simulink subsystem "dq_Limiter"  (R2022b)
settings: Solver=VariableStepAuto  StartTime=0.0  StopTime=10.0  RelTol=1e-3
model mask{X_dq_max=1, limType=Constant ratio d/q, datatype='double'}
  mask prompts: datatype "Signal data type"
libraries: simulink x5
settings Model: Creator=winkens  LastModifiedBy=winkens
settings SolverCC: AlgebraicLoopSolver=TrustRegion
settings DebuggingCC: UnconnectedInputMsg=warning  UnconnectedOutputMsg=warning  UnconnectedLineMsg=warning  SFMachineParentedDataDiag=warning
settings ModelReferenceCC: EnableRefExpFcnMdlSchedulingChecks=on
settings RTWCC: DLArmComputeVersion=19.05

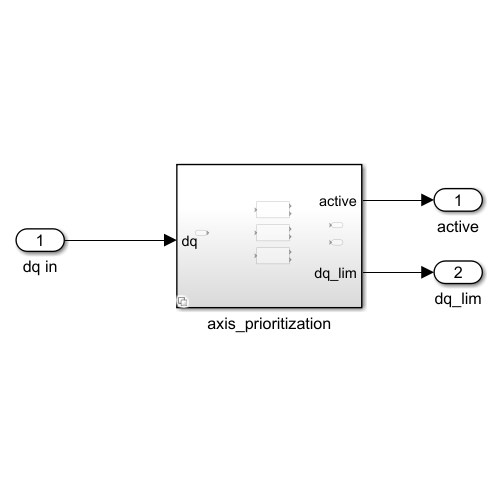
[thumbnail: Simulink's stored preview of the top-level diagram]
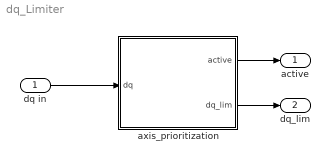
== system dq_Limiter ==
  dq in : Inport
  axis_prioritization : Subsystem  Variant=on
  active : Outport
  dq_lim : Outport  Port=2
  wires:
  dq in/1 -> axis_prioritization/1(dq)
  axis_prioritization/2(dq_lim) -> dq_lim/1
  axis_prioritization/1(active) -> active/1

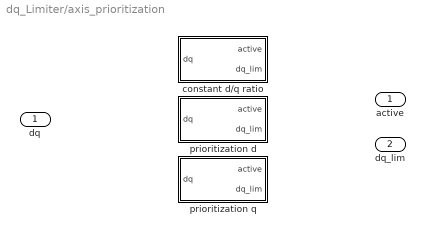
== system dq_Limiter/axis_prioritization ==
  dq : Inport
  constant d/q ratio : Subsystem  VariantControl=(default)
  prioritization d : Subsystem  VariantControl=limType == 2
  prioritization q : Subsystem  VariantControl=limType == 3
  active : Outport  OutDataTypeStr=boolean
  dq_lim : Outport  Port=2

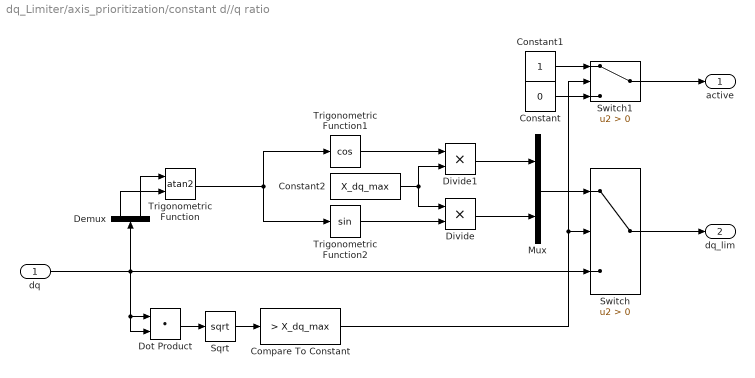
== system dq_Limiter/axis_prioritization/constant d//q ratio ==
  dq : Inport
  Compare To Constant : simulink/Logic and Bit Operations/Compare To Constant  relop=>  const=X_dq_max  OutDataTypeStr=boolean
  Constant : Constant  Value=0  OutDataTypeStr=boolean
  Constant1 : Constant  OutDataTypeStr=boolean
  Constant2 : Constant  Value=X_dq_max  OutDataTypeStr=datatype
  Demux : Demux  Outputs=2
  Divide : Product  Inputs=**
  Divide1 : Product  Inputs=**
  Dot Product : DotProduct  OutDataTypeStr=Inherit: Inherit via internal rule
  Mux : Mux  Inputs=2
  Sqrt : Sqrt
  Switch : Switch  Criteria=u2 > Threshold  SaturateOnIntegerOverflow=off  InputSameDT=off
  Switch1 : Switch  Criteria=u2 > Threshold  SaturateOnIntegerOverflow=off  InputSameDT=off
  Trigonometric Function : Trigonometry  Operator=atan2
  Trigonometric Function1 : Trigonometry  Operator=cos
  Trigonometric Function2 : Trigonometry
  active : Outport  OutDataTypeStr=boolean
  dq_lim : Outport  Port=2
  wires:
  Trigonometric Function/1 -> Trigonometric Function2/1, Trigonometric Function1/1
  Trigonometric Function1/1 -> Divide1/1
  Trigonometric Function2/1 -> Divide/2
  Constant2/1 -> Divide1/2, Divide/1
  Divide/1 -> Mux/2
  Divide1/1 -> Mux/1
  Mux/1 -> Switch/1
  Demux/1 -> Trigonometric Function/2
  Demux/2 -> Trigonometric Function/1
  Compare To Constant/1 -> Switch/2, Switch1/2
  Dot Product/1 -> Sqrt/1
  Switch1/1 -> active/1
  Constant1/1 -> Switch1/1
  Constant/1 -> Switch1/3
  Sqrt/1 -> Compare To Constant/1
  Switch/1 -> dq_lim/1
  dq/1 -> Demux/1, Switch/3, Dot Product/2, Dot Product/1

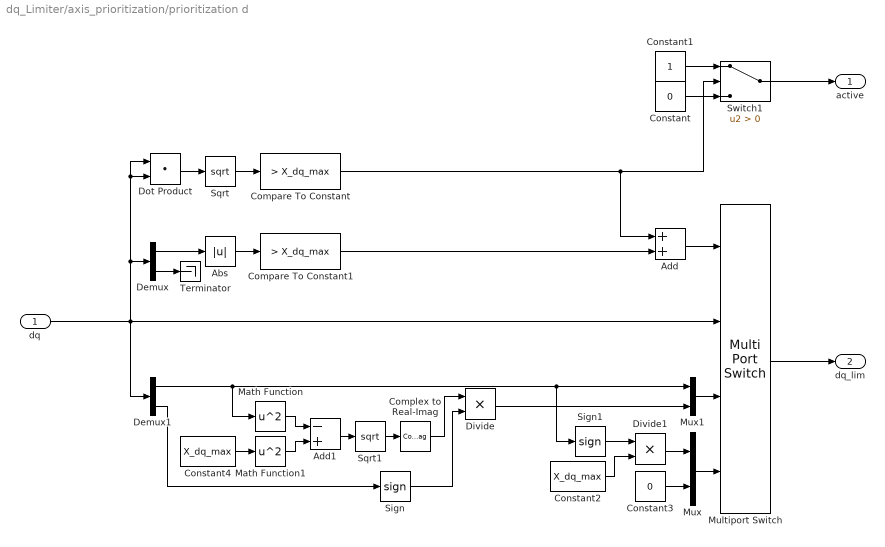
== system dq_Limiter/axis_prioritization/prioritization d ==
  dq : Inport
  Abs : Abs  SaturateOnIntegerOverflow=off
  Add : Sum
  Add1 : Sum  Inputs=-+
  Compare To Constant : simulink/Logic and Bit Operations/Compare To Constant  relop=>  const=X_dq_max  OutDataTypeStr=uint8
  Compare To Constant1 : simulink/Logic and Bit Operations/Compare To Constant  relop=>  const=X_dq_max  OutDataTypeStr=uint8
  Complex to Real-Imag : ComplexToRealImag  Output=Real
  Constant : Constant  Value=0  OutDataTypeStr=boolean
  Constant1 : Constant  OutDataTypeStr=boolean
  Constant2 : Constant  Value=X_dq_max  OutDataTypeStr=datatype
  Constant3 : Constant  Value=0  OutDataTypeStr=datatype
  Constant4 : Constant  Value=X_dq_max  OutDataTypeStr=datatype
  Demux : Demux  Outputs=2
  Demux1 : Demux  Outputs=2
  Divide : Product  Inputs=**
  Divide1 : Product  Inputs=**
  Dot Product : DotProduct  OutDataTypeStr=Inherit: Inherit via internal rule
  Math Function : Math  Operator=square
  Math Function1 : Math  Operator=square
  Multiport Switch : MultiPortSwitch  DataPortOrder=Zero-based contiguous  zeroidx=on  SaturateOnIntegerOverflow=off  InputSameDT=off
  Mux : Mux  Inputs=2
  Mux1 : Mux  Inputs=2
  Sign : Signum
  Sign1 : Signum
  Sqrt : Sqrt
  Sqrt1 : Sqrt  OutputSignalType=complex
  Switch1 : Switch  Criteria=u2 > Threshold  SaturateOnIntegerOverflow=off  InputSameDT=off
  Terminator : Terminator
  active : Outport  OutDataTypeStr=boolean
  dq_lim : Outport  Port=2
  wires:
  Sign1/1 -> Divide1/1
  Constant2/1 -> Divide1/2
  Abs/1 -> Compare To Constant1/1
  Complex to Real-Imag/1 -> Divide/1
  Sqrt1/1 -> Complex to Real-Imag/1
  Sign/1 -> Divide/2
  Divide/1 -> Mux1/2
  Add1/1 -> Sqrt1/1
  Math Function1/1 -> Add1/2
  Math Function/1 -> Add1/1
  Constant4/1 -> Math Function1/1
  Demux1/2 -> Sign/1
  Demux1/1 -> Mux1/1, Sign1/1, Math Function/1
  Mux1/1 -> Multiport Switch/3
  Mux/1 -> Multiport Switch/4
  Constant3/1 -> Mux/2
  Divide1/1 -> Mux/1
  Compare To Constant1/1 -> Add/2
  Add/1 -> Multiport Switch/1
  Demux/1 -> Abs/1
  Demux/2 -> Terminator/1
  Compare To Constant/1 -> Switch1/2, Add/1
  Dot Product/1 -> Sqrt/1
  Switch1/1 -> active/1
  Constant1/1 -> Switch1/1
  Constant/1 -> Switch1/3
  Sqrt/1 -> Compare To Constant/1
  Multiport Switch/1 -> dq_lim/1
  dq/1 -> Multiport Switch/2, Demux/1, Dot Product/2, Dot Product/1, Demux1/1

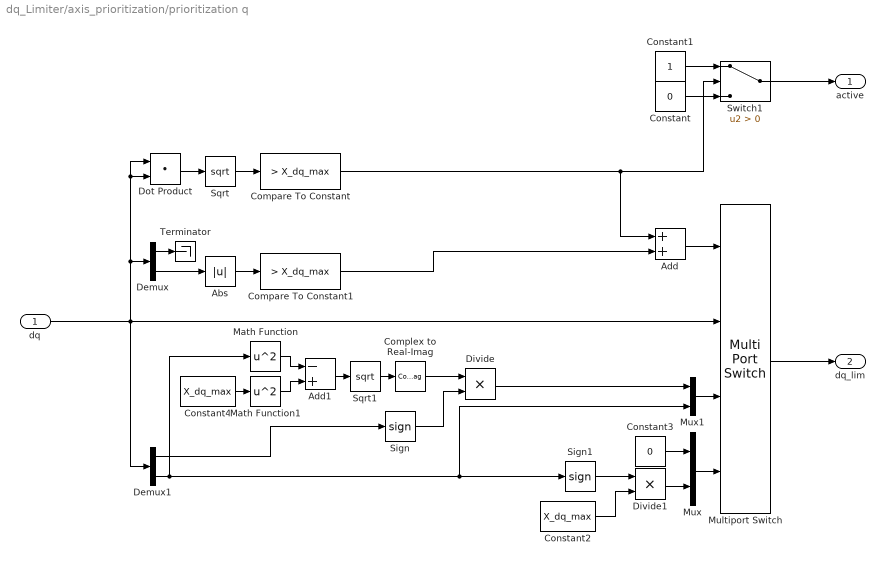
== system dq_Limiter/axis_prioritization/prioritization q ==
  dq : Inport
  Abs : Abs  SaturateOnIntegerOverflow=off
  Add : Sum
  Add1 : Sum  Inputs=-+
  Compare To Constant : simulink/Logic and Bit Operations/Compare To Constant  relop=>  const=X_dq_max  OutDataTypeStr=uint8
  Compare To Constant1 : simulink/Logic and Bit Operations/Compare To Constant  relop=>  const=X_dq_max  OutDataTypeStr=uint8
  Complex to Real-Imag : ComplexToRealImag  Output=Real
  Constant : Constant  Value=0  OutDataTypeStr=boolean
  Constant1 : Constant  OutDataTypeStr=boolean
  Constant2 : Constant  Value=X_dq_max  OutDataTypeStr=datatype
  Constant3 : Constant  Value=0  OutDataTypeStr=datatype
  Constant4 : Constant  Value=X_dq_max  OutDataTypeStr=datatype
  Demux : Demux  Outputs=2
  Demux1 : Demux  Outputs=2
  Divide : Product  Inputs=**
  Divide1 : Product  Inputs=**
  Dot Product : DotProduct  OutDataTypeStr=Inherit: Inherit via internal rule
  Math Function : Math  Operator=square
  Math Function1 : Math  Operator=square
  Multiport Switch : MultiPortSwitch  DataPortOrder=Zero-based contiguous  zeroidx=on  SaturateOnIntegerOverflow=off  InputSameDT=off
  Mux : Mux  Inputs=2
  Mux1 : Mux  Inputs=2
  Sign : Signum
  Sign1 : Signum
  Sqrt : Sqrt
  Sqrt1 : Sqrt  OutputSignalType=complex
  Switch1 : Switch  Criteria=u2 > Threshold  SaturateOnIntegerOverflow=off  InputSameDT=off
  Terminator : Terminator
  active : Outport  OutDataTypeStr=boolean
  dq_lim : Outport  Port=2
  wires:
  Sign1/1 -> Divide1/1
  Constant2/1 -> Divide1/2
  Divide1/1 -> Mux/2
  Abs/1 -> Compare To Constant1/1
  Complex to Real-Imag/1 -> Divide/1
  Sqrt1/1 -> Complex to Real-Imag/1
  Demux1/2 -> Mux1/2, Sign1/1, Math Function/1
  Constant3/1 -> Mux/1
  Sign/1 -> Divide/2
  Divide/1 -> Mux1/1
  Add1/1 -> Sqrt1/1
  Math Function1/1 -> Add1/2
  Math Function/1 -> Add1/1
  Constant4/1 -> Math Function1/1
  Demux1/1 -> Sign/1
  Mux1/1 -> Multiport Switch/3
  Mux/1 -> Multiport Switch/4
  Compare To Constant1/1 -> Add/2
  Add/1 -> Multiport Switch/1
  Demux/1 -> Terminator/1
  Demux/2 -> Abs/1
  Compare To Constant/1 -> Switch1/2, Add/1
  Dot Product/1 -> Sqrt/1
  Switch1/1 -> active/1
  Constant1/1 -> Switch1/1
  Constant/1 -> Switch1/3
  Sqrt/1 -> Compare To Constant/1
  Multiport Switch/1 -> dq_lim/1
  dq/1 -> Multiport Switch/2, Demux/1, Dot Product/2, Dot Product/1, Demux1/1
